simulink model "C6_Word_ClosedLoop_Capture"  (R2025b)
settings: Solver=FixedStepDiscrete  StartTime=0.0  StopTime=120  FixedStep=0.005  RelTol=1e-3
libraries: modelsimlib x1
settings Model: Creator=李晨光  LastModifiedBy=李晨光
settings DataIOCC: SignalLogging=off
settings DebuggingCC: AlgebraicLoopMsg=error

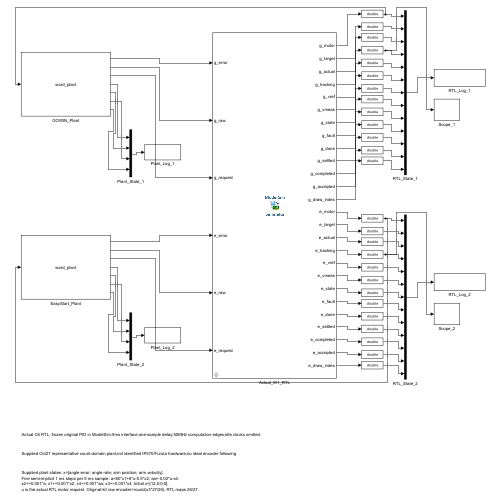
[thumbnail: Simulink's stored preview of the top-level diagram]
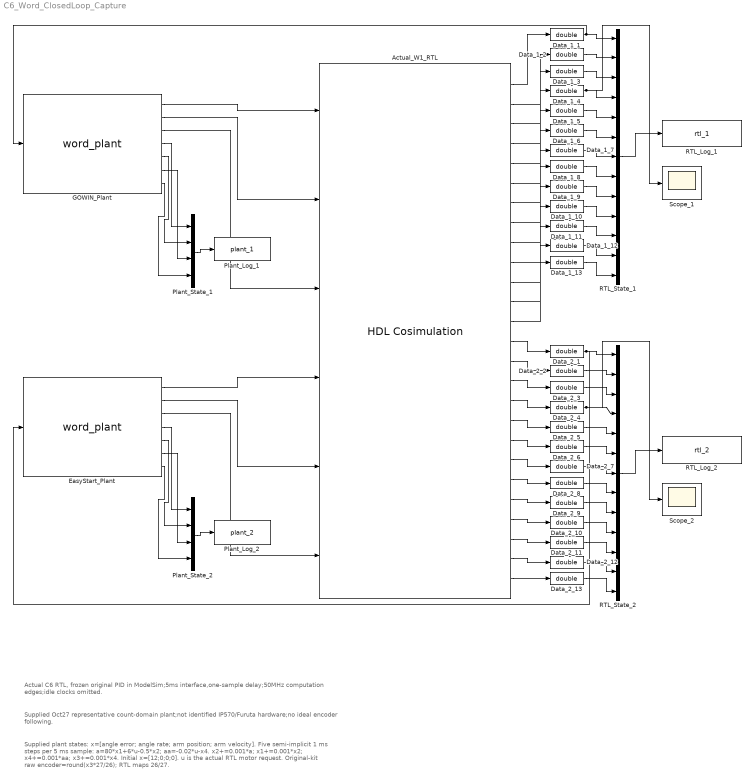
== system C6_Word_ClosedLoop_Capture ==
  note: Actual C6 RTL, frozen original PID in ModelSim;5ms interface,one-sample delay;50MHz computation edges;idle clocks omitted.
  note: Supplied Oct27 representative count-domain plant;not identified IP570/Furuta hardware;no ideal encoder following.
  note: Supplied plant states: x=[angle error; angle rate; arm position; arm velocity].
      | Five semi-implicit 1 ms steps per 5 ms sample: a=80*x1+6*u-0.5*x2; aa=-0.02*u-x4.
      | x2+=0.001*a; x1+=0.001*x2; x4+=0.001*aa; x3+=0.001*x4. Initial x=[12;0;0;0].
      | u is the actual RTL motor request. Original-kit raw encoder=round(x3*27/26); RTL maps 26/27.
  Actual_W1_RTL : modelsimlib/HDL Cosimulation  PortPaths=/word_closed_loop/g_error;/word_closed_loop/g_raw;/word_closed_loop/g_request;/word_closed_loop/e_error;/word_closed_loop/e_raw;/word_closed_loop/e_request;/word_closed_loop/g_motor;/word_closed_loop/g_target;/word_closed_loop/g_actual;/word_closed_loop/g_tracking;/word_closed_loop/g_vref;/word_closed_loop/g_vmeas;/word_closed_loop/g_state;/word_closed_loop/g_fault;/word_closed_loop/g_done;/word_closed_loop/g_settled;/word_closed_loop/g_completed;/word_closed_loop/g_accepted;/word_closed_loop/g_draw_index;/word_closed_loop/e_motor;/word_closed_loop/e_target;/word_closed_loop/e_actual;/word_closed_loop/e_tracking;/word_closed_loop/e_vref;/word_closed_loop/e_vmeas;/word_closed_loop/e_state;/word_closed_loop/e_fault;/word_closed_loop/e_done;/word_closed_loop/e_settled;/word_closed_loop/e_completed;/word_closed_loop/e_accepted;/word_closed_loop/e_draw_index  PortModes=[1 1 1 1 1 1 2 2 2 2 2 2 2 2 2 2 2 2 2 2 2 2 2 2 2 2 2 2 2 2 2 2]  PortTimes=[-1 -1 -1 -1 -1 -1 0.005 0.005 0.005 0.005 0.005 0.005 0.005 0.005 0.005 0.005 0.005 0.005 0.005 0.005 0.005 0.005 0.005 0.005 0.005 0.005 0.005 0.005 0.005 0.005 0.005 0.005]  PortSigns=[-1 -1 -1 -1 -1 -1 1 1 1 1 1 1 0 0 0 0 0 0 0 1 1 1 1 1 1 0 0 0 0 0 0 0]  PortFracLengths=[0 0 0 0 0 0 0 0 0 0 0 0 0 0 0 0 0 0 0 0 0 0 0 0 0 0 0 0 0 0 0 0]  PortWordLengths=[-1 -1 -1 -1 -1 -1 -1 -1 -1 -1 -1 -1 -1 -1 -1 -1 -1 -1 -1 -1 -1 -1 -1 -1 -1 -1 -1 -1 -1 -1 -1 -1]  PortHDLWordSizes=[0 0 0 0 0 0 0 0 0 0 0 0 0 0 0 0 0 0 0 0 0 0 0 0 0 0 0 0 0 0 0 0]  CommLocal=on  CommSharedMemory=off  CommPortNumber=4478  CommShowInfo=off  ClockModes=[]  ClockTimes=[]  TclPreSimCommand=puts {WORD_RUN_STARTED C6 input correction with original PID}  TclPostSimCommand=dataset save sim results/word_font2.wlf; puts {WORD_RUN_FINISHED}  TimingMode=Tick  TimingScaleFactor=1e9  idxCellArray={'UNUSED_VAR'}  CosimBypass=Full Simulation  AllowDirectFeedthrough=off  ProductName=EDA Simulator Link MQ  RunAutoTimescale=off  HdlClocks=0  PreRunTime=0  PreRunTimeUnit=ns
  Data_1_{1..13} (13 alike) : DataTypeConversion  OutDataTypeStr=double  SaturateOnIntegerOverflow=off  RndMeth=Floor
  Data_2_{1..13} (13 alike) : DataTypeConversion  OutDataTypeStr=double  SaturateOnIntegerOverflow=off  RndMeth=Floor
  EasyStart_Plant : M-S-Function  FunctionName=word_plant  Parameters=12
  GOWIN_Plant : M-S-Function  FunctionName=word_plant  Parameters=12
  Plant_Log_1 : ToWorkspace  VariableName=plant_1  SaveFormat=Timeseries  SampleTime=-1
  Plant_Log_2 : ToWorkspace  VariableName=plant_2  SaveFormat=Timeseries  SampleTime=-1
  Plant_State_1 : Mux
  Plant_State_2 : Mux
  RTL_Log_1 : ToWorkspace  VariableName=rtl_1  SaveFormat=Timeseries  SampleTime=-1
  RTL_Log_2 : ToWorkspace  VariableName=rtl_2  SaveFormat=Timeseries  SampleTime=-1
  RTL_State_1 : Mux  Inputs=13
  RTL_State_2 : Mux  Inputs=13
  Scope_1 : Scope
  Scope_2 : Scope
  wires:
  GOWIN_Plant/1 -> Actual_W1_RTL/1
  GOWIN_Plant/2 -> Actual_W1_RTL/2
  GOWIN_Plant/3 -> Actual_W1_RTL/3
  Actual_W1_RTL/1 -> Data_1_1/1
  Actual_W1_RTL/2 -> Data_1_2/1
  Actual_W1_RTL/3 -> Data_1_3/1
  Actual_W1_RTL/4 -> Data_1_4/1
  Actual_W1_RTL/5 -> Data_1_5/1
  Actual_W1_RTL/6 -> Data_1_6/1
  Actual_W1_RTL/7 -> Data_1_7/1
  Actual_W1_RTL/8 -> Data_1_8/1
  Actual_W1_RTL/9 -> Data_1_9/1
  Actual_W1_RTL/10 -> Data_1_10/1
  Actual_W1_RTL/11 -> Data_1_11/1
  Actual_W1_RTL/12 -> Data_1_12/1
  Actual_W1_RTL/13 -> Data_1_13/1
  Data_1_1/1 -> GOWIN_Plant/1, RTL_State_1/1
  GOWIN_Plant/4 -> Plant_State_1/1
  GOWIN_Plant/5 -> Plant_State_1/2
  GOWIN_Plant/6 -> Plant_State_1/3
  GOWIN_Plant/7 -> Plant_State_1/4
  Plant_State_1/1 -> Plant_Log_1/1
  Data_1_2/1 -> RTL_State_1/2
  Data_1_3/1 -> RTL_State_1/3
  Data_1_4/1 -> RTL_State_1/4, Scope_1/1
  Data_1_5/1 -> RTL_State_1/5
  Data_1_6/1 -> RTL_State_1/6
  Data_1_7/1 -> RTL_State_1/7
  Data_1_8/1 -> RTL_State_1/8
  Data_1_9/1 -> RTL_State_1/9
  Data_1_10/1 -> RTL_State_1/10
  Data_1_11/1 -> RTL_State_1/11
  Data_1_12/1 -> RTL_State_1/12
  Data_1_13/1 -> RTL_State_1/13
  RTL_State_1/1 -> RTL_Log_1/1
  EasyStart_Plant/1 -> Actual_W1_RTL/4
  EasyStart_Plant/2 -> Actual_W1_RTL/5
  EasyStart_Plant/3 -> Actual_W1_RTL/6
  Actual_W1_RTL/14 -> Data_2_1/1
  Actual_W1_RTL/15 -> Data_2_2/1
  Actual_W1_RTL/16 -> Data_2_3/1
  Actual_W1_RTL/17 -> Data_2_4/1
  Actual_W1_RTL/18 -> Data_2_5/1
  Actual_W1_RTL/19 -> Data_2_6/1
  Actual_W1_RTL/20 -> Data_2_7/1
  Actual_W1_RTL/21 -> Data_2_8/1
  Actual_W1_RTL/22 -> Data_2_9/1
  Actual_W1_RTL/23 -> Data_2_10/1
  Actual_W1_RTL/24 -> Data_2_11/1
  Actual_W1_RTL/25 -> Data_2_12/1
  Actual_W1_RTL/26 -> Data_2_13/1
  Data_2_1/1 -> EasyStart_Plant/1, RTL_State_2/1
  EasyStart_Plant/4 -> Plant_State_2/1
  EasyStart_Plant/5 -> Plant_State_2/2
  EasyStart_Plant/6 -> Plant_State_2/3
  EasyStart_Plant/7 -> Plant_State_2/4
  Plant_State_2/1 -> Plant_Log_2/1
  Data_2_2/1 -> RTL_State_2/2
  Data_2_3/1 -> RTL_State_2/3
  Data_2_4/1 -> RTL_State_2/4, Scope_2/1
  Data_2_5/1 -> RTL_State_2/5
  Data_2_6/1 -> RTL_State_2/6
  Data_2_7/1 -> RTL_State_2/7
  Data_2_8/1 -> RTL_State_2/8
  Data_2_9/1 -> RTL_State_2/9
  Data_2_10/1 -> RTL_State_2/10
  Data_2_11/1 -> RTL_State_2/11
  Data_2_12/1 -> RTL_State_2/12
  Data_2_13/1 -> RTL_State_2/13
  RTL_State_2/1 -> RTL_Log_2/1
